simulink model "dual_yaw_lqr"  (R2024a)
settings: Solver=ode4  StartTime=0.0  StopTime=p.stop_time  FixedStep=p.solver_step  RelTol=1e-3
model workspace (MAT data in the model file):
  p.model_mode = 'article'
  p.controller_mode = 'continuous'
  p.parameter_note = 'J1/J2: article CAD estimates, not identified values. Limits and 1-ms step: article settings. B1/B2: unknown, zero assumption. Q/R and waveform parameters: demonstration values, not original tuning.'
  p.source_url = 'https://bbs.robomaster.com/wiki/36827278/1647282?source=7#head8'
  p.J1 = 0.178592
  p.J2 = 0.044374
  p.B1 = 0
  p.B2 = 0
  p.Ts = 0.001
  p.solver_step = 0.001
  p.stop_time = 10
  p.torque_limit = [7; 1.2]
  p.dead_zone = [0; 0]
  p.Q = [120  0  0  0; 0  1.5  0  0; 0  0  300  0; 0  0  0  2]
  p.R = [1  0; 0  0.6]
  p.x0 = [0; 0; 0; 0]
  p.enable_feedforward = 0
  p.ref_kind = 'article'
  p.ref_amplitude = 0.261799387799
  p.ref_f1 = 0.5
  p.ref_f2 = 1
  p.ref_big_ratio = 1
  p.ref_start = 1
  p.ref_ramp = 0.5
  p.ref_reset_ratio = 0.2
  p.M = [0.222966  0.044374; 0.044374  0.044374]
  p.A = [0  1  0  0; 0  0  0  0; 0  0  0  1; 0  0  0  0]
  p.B = [0  0; 5.59935495431  -5.59935495431; 0  0; -5.59935495431  28.1350740691]
  p.coordinate_system = 'big_absolute_small_relative'
  p.C = [1  0  0  0; 0  1  0  0; 0  0  1  0; 0  0  0  1]
  p.D = [0  0; 0  0; 0  0; 0  0]
  p.controllability_rank = 4
  p.Ad = []
  p.Bd = []
  p.K = [10.9535526986  2.519709192  -0.221829212769  0.262753073282; 0.181122793776  0.274620408174  22.3588458185  2.27371048902]
  p.riccati_solution = [27.6296114289  2.4470921167  3.1251721125  0.490875233157; 2.4470921167  0.569121083299  0.545830482355  0.119121179281; 3.1251721125  0.545830482355  30.4442390485  0.585447405122; 0.490875233157  0.119121179281  0.585447405122  0.0721955824176]
  p.closed_loop_poles = [-5.5894460126+4.11067562324i; -5.5894460126-4.11067562324i; -12.4915624039+0i; -51.4003598731+0i]
  p.sample_time = 0
  u_ff_input = timeseries
  u_ff_input.Name = 'unnamed'
  u_ff_input.DataInfo = tsdata.datametadata
  u_ff_input.DataInfo.Interpolation = tsdata.interpolation
  u_ff_input.DataInfo.Interpolation.Fhandle : function handle (value not decoded)
  u_ff_input.DataInfo.Interpolation.Name = 'linear'
  u_ff_input.TimeInfo = tsdata.timemetadata
  u_ff_input.TimeInfo.Length = 10001
  u_ff_input.TimeInfo.DuplicateTimes = 0
  u_ff_input.TimeInfo.Time_ = [0 0.001 0.002 0.003 0.004 0.005 0.006 0.007 0.008 0.009 0.01 0.011 ... (10001 elements, 10001x1)]
  u_ff_input.TimeInfo.Initialized = 1
  u_ff_input.QualityInfo = tsdata.qualmetadata
  u_ff_input.Data_ = [0 0 0 0 0 0 0 0 0 0 0 0 ... (20002 elements, 10001x2)]
  x_ref_input = timeseries
  x_ref_input.Name = 'unnamed'
  x_ref_input.DataInfo = tsdata.datametadata
  x_ref_input.DataInfo.Interpolation = tsdata.interpolation
  x_ref_input.DataInfo.Interpolation.Fhandle : function handle (value not decoded)
  x_ref_input.DataInfo.Interpolation.Name = 'linear'
  x_ref_input.TimeInfo = tsdata.timemetadata
  x_ref_input.TimeInfo.Length = 10001
  x_ref_input.TimeInfo.DuplicateTimes = 0
  x_ref_input.TimeInfo.Time_ = [0 0.001 0.002 0.003 0.004 0.005 0.006 0.007 0.008 0.009 0.01 0.011 ... (10001 elements, 10001x1)]
  x_ref_input.TimeInfo.Initialized = 1
  x_ref_input.QualityInfo = tsdata.qualmetadata
  x_ref_input.Data_ = [0 0 0 0 0 0 0 0 0 0 0 0 ... (40004 elements, 10001x4)]
values from neighbouring files (symbols this model uses):
  p = dual_yaw_parameters()    [build_dual_yaw_lqr.m]    (also in dual_yaw_configure.m = dual_yaw_design(p); dual_yaw_parameters.m = dual_yaw_design(p); run_dual_yaw_lqr.m = dual_yaw_configure(model, p); validate_dual_yaw_lqr.m)
settings Model: Creator=m6jia  LastModifiedBy=m6jia
settings DataIOCC: SaveOutput=off  SignalLogging=off

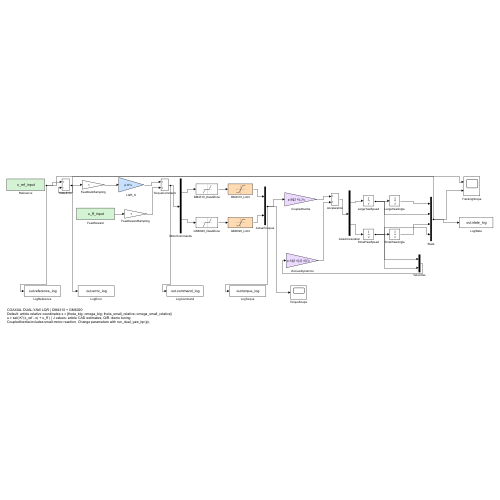
[thumbnail: Simulink's stored preview of the top-level diagram]
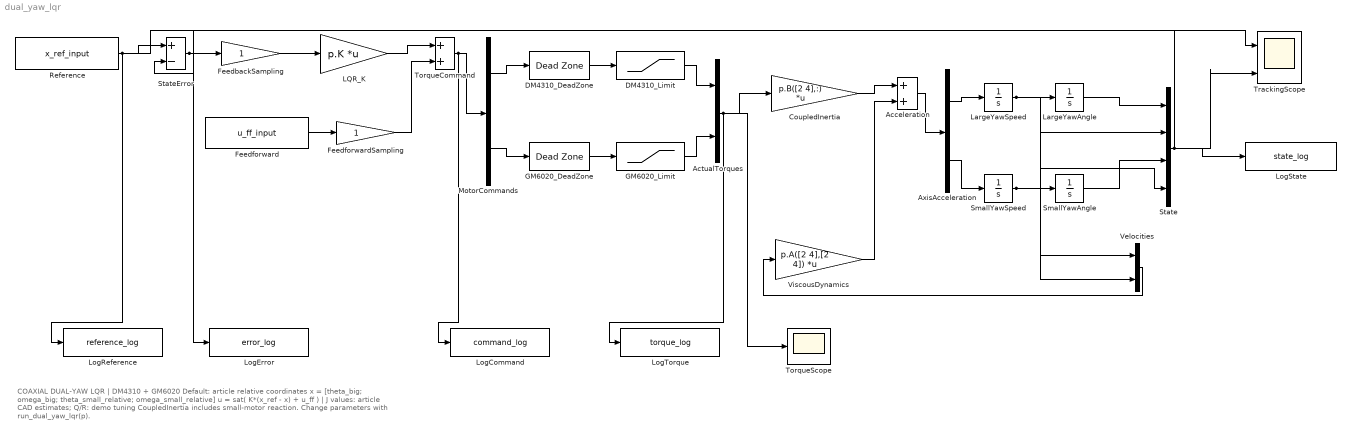
== system dual_yaw_lqr ==
  note: COAXIAL DUAL-YAW LQR | DM4310 + GM6020
      | Default: article relative coordinates x = [theta_big; omega_big; theta_small_relative; omega_small_relative]
      | u = sat( K*(x_ref - x) + u_ff ) | J values: article CAD estimates; Q/R: demo tuning
      | CoupledInertia includes small-motor reaction. Change parameters with run_dual_yaw_lqr(p).
  Acceleration : Sum
  ActualTorques : Mux  Inputs=2
  AxisAcceleration : Demux  Outputs=2
  CoupledInertia : Gain  Gain=p.B([2 4],:)  Multiplication=Matrix(K*u)
  DM4310_DeadZone : DeadZone  LowerValue=-p.dead_zone(1)  UpperValue=p.dead_zone(1)
  DM4310_Limit : Saturate  UpperLimit=p.torque_limit(1)  LowerLimit=-p.torque_limit(1)
  FeedbackSampling : Gain
  Feedforward : FromWorkspace  VariableName=u_ff_input
  FeedforwardSampling : Gain
  GM6020_DeadZone : DeadZone  LowerValue=-p.dead_zone(2)  UpperValue=p.dead_zone(2)
  GM6020_Limit : Saturate  UpperLimit=p.torque_limit(2)  LowerLimit=-p.torque_limit(2)
  LQR_K : Gain  Gain=p.K  Multiplication=Matrix(K*u)
  LargeYawAngle : Integrator  InitialCondition=p.x0(1)
  LargeYawSpeed : Integrator  InitialCondition=p.x0(2)
  LogCommand : ToWorkspace  VariableName=command_log  SaveFormat=Timeseries  SampleTime=-1
  LogError : ToWorkspace  VariableName=error_log  SaveFormat=Timeseries  SampleTime=-1
  LogReference : ToWorkspace  VariableName=reference_log  SaveFormat=Timeseries  SampleTime=-1
  LogState : ToWorkspace  VariableName=state_log  SaveFormat=Timeseries  SampleTime=-1
  LogTorque : ToWorkspace  VariableName=torque_log  SaveFormat=Timeseries  SampleTime=-1
  MotorCommands : Demux  Outputs=2
  Reference : FromWorkspace  VariableName=x_ref_input
  SmallYawAngle : Integrator  InitialCondition=p.x0(3)
  SmallYawSpeed : Integrator  InitialCondition=p.x0(4)
  State : Mux
  StateError : Sum  Inputs=+-
  TorqueCommand : Sum
  TorqueScope : Scope
  TrackingScope : Scope  NumInputPorts=2
  Velocities : Mux  Inputs=2
  ViscousDynamics : Gain  Gain=p.A([2 4],[2 4])  Multiplication=Matrix(K*u)
  wires:
  Reference/1 -> StateError/1, TrackingScope/1, LogReference/1
  State/1 -> StateError/2, TrackingScope/2, LogState/1
  StateError/1 -> FeedbackSampling/1, LogError/1
  FeedbackSampling/1 -> LQR_K/1
  LQR_K/1 -> TorqueCommand/1
  Feedforward/1 -> FeedforwardSampling/1
  FeedforwardSampling/1 -> TorqueCommand/2
  TorqueCommand/1 -> MotorCommands/1, LogCommand/1
  MotorCommands/1 -> DM4310_DeadZone/1
  DM4310_DeadZone/1 -> DM4310_Limit/1
  MotorCommands/2 -> GM6020_DeadZone/1
  GM6020_DeadZone/1 -> GM6020_Limit/1
  DM4310_Limit/1 -> ActualTorques/1
  GM6020_Limit/1 -> ActualTorques/2
  ActualTorques/1 -> CoupledInertia/1, LogTorque/1, TorqueScope/1
  CoupledInertia/1 -> Acceleration/1
  ViscousDynamics/1 -> Acceleration/2
  Acceleration/1 -> AxisAcceleration/1
  AxisAcceleration/1 -> LargeYawSpeed/1
  LargeYawSpeed/1 -> LargeYawAngle/1, Velocities/1, State/2
  AxisAcceleration/2 -> SmallYawSpeed/1
  SmallYawSpeed/1 -> SmallYawAngle/1, Velocities/2, State/4
  Velocities/1 -> ViscousDynamics/1
  LargeYawAngle/1 -> State/1
  SmallYawAngle/1 -> State/3
